simulink model "fw_io_in_sim"  (R2026b)
settings: Solver=VariableStepAuto
undefined symbols (not defined in the file or in its folder): Ts
libraries: simulink x4
settings Model: Creator=aomar  LastModifiedBy=aomar

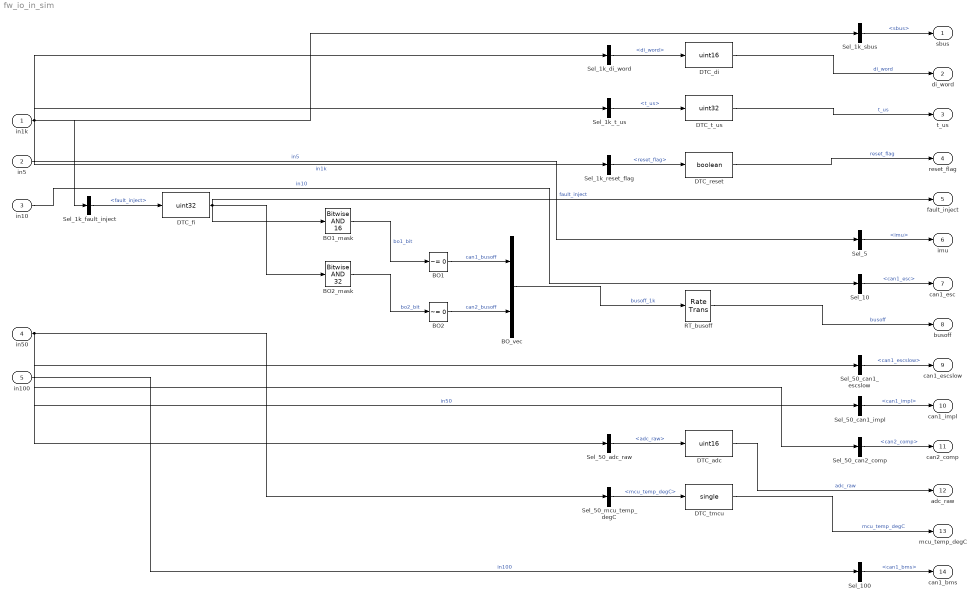
== system fw_io_in_sim ==
  in1k : Inport  OutDataTypeStr=Bus: Bus_McuIn1k  SampleTime=Ts.base
  in5 : Inport  Port=2  OutDataTypeStr=Bus: Bus_McuIn5  SampleTime=Ts.imu
  in10 : Inport  Port=3  OutDataTypeStr=Bus: Bus_McuIn10  SampleTime=Ts.ctrl
  in50 : Inport  Port=4  OutDataTypeStr=Bus: Bus_McuIn50  SampleTime=Ts.comm
  in100 : Inport  Port=5  OutDataTypeStr=Bus: Bus_McuIn100  SampleTime=Ts.hk
  BO1 : simulink/Logic and Bit Operations/Compare To Zero  relop=~=  OutDataTypeStr=boolean
  BO1_mask : simulink/Logic and Bit Operations/Bitwise Operator  logicop=AND  UseBitMask=on  BitMask=16  BitMaskRealWorld=Stored Integer
  BO2 : simulink/Logic and Bit Operations/Compare To Zero  relop=~=  OutDataTypeStr=boolean
  BO2_mask : simulink/Logic and Bit Operations/Bitwise Operator  logicop=AND  UseBitMask=on  BitMask=32  BitMaskRealWorld=Stored Integer
  BO_vec : Concatenate
  DTC_adc : DataTypeConversion  OutDataTypeStr=uint16  RndMeth=Round
  DTC_di : DataTypeConversion  OutDataTypeStr=uint16  RndMeth=Round
  DTC_fi : DataTypeConversion  OutDataTypeStr=uint32  RndMeth=Round
  DTC_reset : DataTypeConversion  OutDataTypeStr=boolean  RndMeth=Round
  DTC_t_us : DataTypeConversion  OutDataTypeStr=uint32  RndMeth=Round
  DTC_tmcu : DataTypeConversion  OutDataTypeStr=single  RndMeth=Round
  RT_busoff : RateTransition  InitialCondition=false  OutPortSampleTime=Ts.ctrl
  Sel_10 : BusSelector  OutputSignals=can1_esc
  Sel_100 : BusSelector  OutputSignals=can1_bms
  Sel_1k_di_word : BusSelector  OutputSignals=di_word
  Sel_1k_fault_inject : BusSelector  OutputSignals=fault_inject
  Sel_1k_reset_flag : BusSelector  OutputSignals=reset_flag
  Sel_1k_sbus : BusSelector  OutputSignals=sbus
  Sel_1k_t_us : BusSelector  OutputSignals=t_us
  Sel_5 : BusSelector  OutputSignals=imu
  Sel_50_adc_raw : BusSelector  OutputSignals=adc_raw
  Sel_50_can1_escslow : BusSelector  OutputSignals=can1_escslow
  Sel_50_can1_impl : BusSelector  OutputSignals=can1_impl
  Sel_50_can2_comp : BusSelector  OutputSignals=can2_comp
  Sel_50_mcu_temp_degC : BusSelector  OutputSignals=mcu_temp_degC
  sbus : Outport  OutDataTypeStr=Bus: Bus_SbusStream
  di_word : Outport  Port=2  OutDataTypeStr=uint16
  t_us : Outport  Port=3  OutDataTypeStr=uint32
  reset_flag : Outport  Port=4  OutDataTypeStr=boolean
  fault_inject : Outport  Port=5  OutDataTypeStr=uint32
  imu : Outport  Port=6  OutDataTypeStr=Bus: Bus_ImuRaw
  can1_esc : Outport  Port=7  OutDataTypeStr=Bus: Bus_Can1_EscFast
  busoff : Outport  Port=8  OutDataTypeStr=boolean
  can1_escslow : Outport  Port=9  OutDataTypeStr=Bus: Bus_Can1_EscSlow
  can1_impl : Outport  Port=10  OutDataTypeStr=Bus: Bus_Can1_Impl
  can2_comp : Outport  Port=11  OutDataTypeStr=Bus: Bus_CanFrame64
  adc_raw : Outport  Port=12  OutDataTypeStr=uint16
  mcu_temp_degC : Outport  Port=13  OutDataTypeStr=single
  can1_bms : Outport  Port=14  OutDataTypeStr=Bus: Bus_Can1_Bms
  wires:
  in5/1 -> Sel_5/1  "in5"
  in50/1 -> Sel_50_mcu_temp_degC/1, Sel_50_can2_comp/1, Sel_50_adc_raw/1, Sel_50_can1_impl/1, Sel_50_can1_escslow/1  "in50"
  in100/1 -> Sel_100/1  "in100"
  Sel_1k_fault_inject/1 -> DTC_fi/1  "<fault_inject>"
  DTC_fi/1 -> BO2_mask/1, BO1_mask/1, fault_inject/1  "fault_inject"
  BO1_mask/1 -> BO1/1  "bo1_bit"
  BO2_mask/1 -> BO2/1  "bo2_bit"
  BO1/1 -> BO_vec/1  "can1_busoff"
  BO2/1 -> BO_vec/2  "can2_busoff"
  BO_vec/1 -> RT_busoff/1  "busoff_1k"
  Sel_1k_di_word/1 -> DTC_di/1  "<di_word>"
  Sel_1k_t_us/1 -> DTC_t_us/1  "<t_us>"
  Sel_1k_reset_flag/1 -> DTC_reset/1  "<reset_flag>"
  Sel_50_adc_raw/1 -> DTC_adc/1  "<adc_raw>"
  Sel_50_mcu_temp_degC/1 -> DTC_tmcu/1  "<mcu_temp_degC>"
  RT_busoff/1 -> busoff/1  "busoff"
  DTC_di/1 -> di_word/1  "di_word"
  DTC_t_us/1 -> t_us/1  "t_us"
  DTC_reset/1 -> reset_flag/1  "reset_flag"
  DTC_adc/1 -> adc_raw/1  "adc_raw"
  DTC_tmcu/1 -> mcu_temp_degC/1  "mcu_temp_degC"
  Sel_1k_sbus/1 -> sbus/1  "<sbus>"
  Sel_5/1 -> imu/1  "<imu>"
  Sel_10/1 -> can1_esc/1  "<can1_esc>"
  Sel_50_can1_escslow/1 -> can1_escslow/1  "<can1_escslow>"
  Sel_50_can1_impl/1 -> can1_impl/1  "<can1_impl>"
  Sel_50_can2_comp/1 -> can2_comp/1  "<can2_comp>"
  Sel_100/1 -> can1_bms/1  "<can1_bms>"
  in1k/1 -> Sel_1k_sbus/1, Sel_1k_fault_inject/1, Sel_1k_di_word/1, Sel_1k_reset_flag/1, Sel_1k_t_us/1  "in1k"
  in10/1 -> Sel_10/1  "in10"
